simulink model "hydelcompleted_nosubsys"  (R2024b)
settings: Solver=VariableStepAuto  StartTime=0.0  StopTime=10.0  RelTol=1e-3
libraries: spsLoadFlowBusLib x3, spsThreePhaseParallelRLCLoadLib x2, spsThreePhaseVIMeasurementLib x2, spsDistributedParametersLineLib x1, spsExcitationSystemLib x1, spsHydraulicTurbineandGovernorLib x1, spsPower3phInstantaneousLib x1, spsSynchronousMachinepuStandardLib x1, spsThreePhaseTransformerTwoWindingsLib x1, sps_lib x1
settings Model: Creator=Ram  LastModifiedBy=Ram

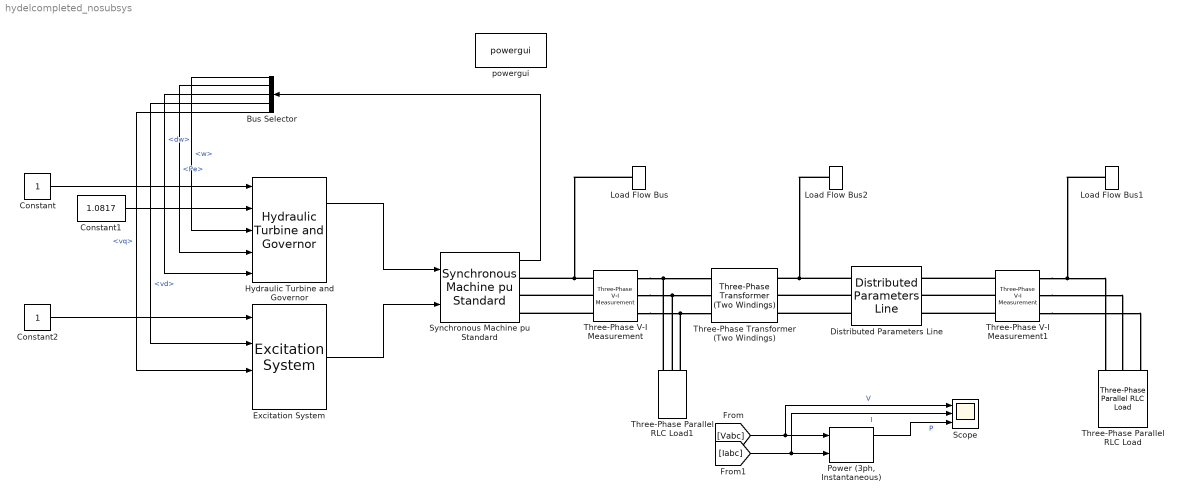
== system hydelcompleted_nosubsys ==
  Bus Selector : BusSelector  OutputSignals=w,Pe,dw,vd,vq
  Constant : Constant
  Constant1 : Constant  Value=1.0817
  Constant2 : Constant
  Distributed Parameters Line : spsDistributedParametersLineLib/Distributed Parameters Line  Phases=3  Length=100  Frequency=50  Resistance=[0.01273 0.3864]  Inductance="[0.9337e-3  4.1264e-3]"  Capacitance=[12.74e-9 7.751e-9]  x1=[-0.0006 -3.40260704829599e-09 112958.573096956 -396382.373244938;-0.00055 -3.37817671582999e-09 119170.741391489 -394559.196384513;-0.0005 -3.35291286880809e-09 125353.506088773 -392638.667946296;-0.00045 -3.32682174070653e-09 131505.341684135 -390621.261791942;-0.0004 -3.29990976912076e-09 137624.730304193 -388507.475686232;-0.00035 -3.27218359417706e-09 143710.162081371 -386297.831174258;-0.0003 -3.24365005689423e-09 149760.135526437 -383992.873452741;-0.00025 -3.21431619749565e-09 155773.157898971 -381593.171235508;-0.0002 -3.18418925367217e-09 161747.745575677 -379099.316613174;-0.00015 -3.1532766587964e-09 167682.424416446 -376511.92490705;-0.0001 -3.12158604008856e-09 173575.730128076 -373831.634517325;-5e-05 -3.08912521673463e-09 179426.208625566 -371059.106765545]  x2=[-0.0006 -3.5386891368581e-09 106068.858641917 -400380.951134164;-0.00055 -3.5176747746853e-09 112344.683835126 -398665.499910241;-0.0005 -3.49579247889795e-09 118592.789658648 -396851.683939575;-0.00045 -3.4730476486251e-09 124811.634485864 -394939.950754116;-0.0004 -3.44944589581327e-09 130999.683909868 -392930.772045422;-0.00035 -3.42499304384182e-09 137155.411122057 -390824.643548275;-0.0003 -3.39969512608608e-09 143277.297288852 -388622.084918367;-0.00025 -3.3735583844287e-09 149363.831926445 -386323.639604083;-0.0002 -3.3465892677196e-09 155413.513273489 -383929.874712411;-0.00015 -3.31879443018478e-09 161424.848661635 -381441.380869019;-0.0001 -3.2901807297845e-09 167396.354883826 -378858.772072529;-5e-05 -3.26075522652118e-09 173326.558560255 -376182.685543014]  x3=[-0.0006 -2.64139611004173e-12 190.415973613975 -1253.14025946932;-0.00055 -2.63703449038585e-12 210.07595415956 -1249.99473854659;-0.0005 -2.63202222192825e-12 229.684101606891 -1246.54080012619;-0.00045 -2.62636054137119e-12 249.235577938987 -1242.77929641575;-0.0004 -2.62005084564962e-12 268.725559121619 -1238.71115551002;-0.00035 -2.61309469158654e-12 288.149236293565 -1234.33738116191;-0.0003 -2.6054937955089e-12 307.501816953124 -1229.65905253478;-0.00025 -2.59725003282405e-12 326.778526140599 -1224.67732393622;-0.0002 -2.58836543755709e-12 345.974607616441 -1219.39342453322;-0.00015 -2.57884220184896e-12 365.085325034782 -1213.80865804889;-0.0001 -2.56868267541556e-12 384.10596311206 -1207.9244024408;-5e-05 -2.55788936496803e-12 403.031828790441 -1201.74210956096]  x4=[-0.0006 -7.19418612714017e-12 456.56208442296 -1723.39809180542;-0.00055 -7.1670537441911e-12 483.57572017421 -1716.01411492715;-0.0005 -7.13815299797357e-12 510.470040852406 -1708.20673724329;-0.00045 -7.10749101931428e-12 537.238410686349 -1699.97788510746;-0.0004 -7.07507537359763e-12 563.874224981325 -1691.32958886579;-0.00035 -7.04091405889918e-12 590.370911748719 -1682.26398235598;-0.0003 -7.00501550401215e-12 616.721933327548 -1672.78330238078;-0.00025 -6.96738856636781e-12 642.920787997537 -1662.88988815611;-0.0002 -6.92804252984998e-12 668.961011583318 -1652.58618073389;-0.00015 -6.88698710250445e-12 694.836179049369 -1641.87472239975;-0.0001 -6.84423241414356e-12 720.539906085297 -1630.75815604577;-5e-05 -6.79978901384694e-12 746.065850681068 -1619.23922451833]  x5=0.000565541566995743  V1=[2.409e-07 4.122e+05 4.122e+05;314.2 314.2 314.2;0.4186 0.3578 -1.213]  V2=[2.389e-07 4.142e+05 4.142e+05;314.2 314.2 314.2;0.3317 0.3391 -1.232]  I1=[1.745e-10 1268 1268;314.2 314.2 314.2;0.1145 0.2309 -1.34]  I2=[4.629e-10 1783 1783;314.2 314.2 314.2;0.3479 0.3391 -1.232]  nHarmo=1  Measurements=None  Decoupling=off  VsMag0=0  VrMag0=0  VsAngle0=0  VrAngle0=0  IsMag0=0  IrMag0=0  IsAngle0=0  IrAngle0=0
      settings: LibrarySourceBlock=sps_lib/Power Grid Elements/Distributed Parameters Line
  Excitation System : spsExcitationSystemLib/Excitation System  tr=20e-3  reg=[ 300, 0.001 ]  exc=[ 1, 0 ]  tgr=[ 0, 0 ]  damp=[ 0.001, 0.1 ]  sat=[ 0, 0 ]  lim=[ -11.5, 11.5, 0 ]  v0=[1 2.1744]
      settings: LibrarySourceBlock=sps_lib/Electrical Machines/Synchronous Machine Control/Excitation System
  Hydraulic Turbine and Governor : spsHydraulicTurbineandGovernorLib/Hydraulic Turbine and Governor  sm="[ 10/3  0.07 ]"  gate="[  0.01  0.97518  -0.1  0.1 ]"  reg="[  0.05  1.163  0.105  0  0.01  ]"  hyd="[  0  2.67  ]"  dref=0  po=1.0094
      settings: LibrarySourceBlock=|
      | sps_lib/Electrical Machines/Synchronous Machine Control/Hydraulic Turbine
      | and Governor
  Load Flow Bus : spsLoadFlowBusLib/Load Flow Bus  LConnTagsString=a  Phases=single  Connectors=on one side  ID=BUS_1  Vbase=13.8e3  Vref=1  Vangle=0  VLF=1  VLFb=1  VLFc=1  angleLF=0  angleLFb=0  angleLFc=0
  Load Flow Bus1 : spsLoadFlowBusLib/Load Flow Bus  LConnTagsString=a  Phases=single  Connectors=on one side  ID=BUS_3  Vbase=400e3  Vref=1  Vangle=0  VLF=1.036  VLFb=1  VLFc=1  angleLF=-4.321  angleLFb=0  angleLFc=0
  Load Flow Bus2 : spsLoadFlowBusLib/Load Flow Bus  LConnTagsString=a  Phases=single  Connectors=on one side  ID=BUS_2  Vbase=400e3  Vref=1  Vangle=0  VLF=1.031  VLFb=1  VLFc=1  angleLF=-3.252  angleLFb=0  angleLFc=0
  "Power (3ph, Instantaneous)" : spsPower3phInstantaneousLib/Power (3ph, Instantaneous)
  Scope : Scope  NumInputPorts=3
  Synchronous Machine pu Standard : spsSynchronousMachinepuStandardLib/Synchronous Machine pu Standard  PresetModel=No  MechanicalLoad=Mechanical power Pm  ShowDetailedParameters=on  RotorType=Salient-pole  Units=per unit standard parameters  MeasurementBus=on  NominalParameters=[100e6 13.8e3 50]  Reactances1=[ 1.81, 0.3, 0.23, 1.76, 0.65, 0.25, 0.15 ]  Reactances2=[2.24 0.17 0.12 1.02 0.13 0.08]  dAxisTimeConstants=Short-circuit  qAxisTimeConstants=Short-circuit  TimeConstants1="[ 4.4849  0.0681  0.1  ]"  TimeConstants2=[ 8.0, 0.03, 1.0, 0.07 ]  TimeConstants3="[  4.49  0.0681  0.0513  ]"  TimeConstants4=[ 8.0, 0.03, 0.3371, 0.0295 ]  TimeConstants5=[ 1.01, 0.053, 0.1 ]  TimeConstants6=[ 1.3201, 0.023, 1.0, 0.07 ]  TimeConstants7=[0.012 0.003 0.003]  TimeConstants8=[ 1.3201, 0.0231, 0.3371, 0.0295 ]  StatorResistance=0.037875  Mechanical=[0.1028 0.02056 12]  PolePairs=20  InitialConditions=[0 -21.9196 1.2258 1.2258 1.2258 28.0638 -91.9362 148.064 2.17443]  SetSaturation=on  Saturation=[0.6404,0.7127,0.8441,0.9214,0.9956,1.082,1.19,1.316,1.457;0.7,0.7698,0.8872,0.9466,0.9969,1.046,1.1,1.151,1.201]  LoadFlowParameters=[1,0,0,0,0]  TsPowergui=0  TsBlock=-1  IterativeModel=Trapezoidal non iterative  IterativeDiscreteModel=Trapezoidal non iterative  BusType=swing  Pref=0  Qref=0  Qmin=-Inf  Qmax=Inf  PLF=0  QLF=0
  Three-Phase Parallel RLC Load : spsThreePhaseParallelRLCLoadLib/Three-Phase Parallel RLC Load  LConnTagsString=A|B|C  Configuration=Y (grounded)  NominalVoltage=400e3  Vabc=[1e3 1e3 1e3]  Vabcp=[1e3 1e3 1e3]  NominalFrequency=50  UnbalancedPower=off  ActivePower=100000000  InductivePower=100  CapacitivePower=0  Pabc=[10e3 9e3 11e3]  QLabc=[100 90 110]  QCabc=[100 90 110]  Pabcp=[10e3 9e3 11e3]  QLabcp=[100 90 110]  QCabcp=[100 90 110]  Measurements=None  LoadType=constant Z
  Three-Phase Parallel RLC Load1 : spsThreePhaseParallelRLCLoadLib/Three-Phase Parallel RLC Load  LConnTagsString=A|B|C  Configuration=Y (grounded)  NominalVoltage=13.8e3  Vabc=[1e3 1e3 1e3]  Vabcp=[1e3 1e3 1e3]  NominalFrequency=50  UnbalancedPower=off  ActivePower=100  InductivePower=0  CapacitivePower=0  Pabc=[10e3 9e3 11e3]  QLabc=[100 90 110]  QCabc=[100 90 110]  Pabcp=[10e3 9e3 11e3]  QLabcp=[100 90 110]  QCabcp=[100 90 110]  Measurements=None  LoadType=constant Z
  Three-Phase Transformer (Two Windings) : spsThreePhaseTransformerTwoWindingsLib/Three-Phase Transformer (Two Windings)  Winding1Connection=Yg  Winding2Connection=Yg  CoreType=Three single-phase transformers  SetSaturation=off  Hysteresis=off  DataFile='hysteresis'  SetInitialFlux=off  Measurements=None  UNITS=pu  NominalPower=[ 250e6 , 50 ]  Winding1=[ 13.8e3 , 0.002 , 0.08 ]  Winding2=[ 400e3 , 0.002 , 0.08 ]  Rm=500  Lm=500  L0=0.5  Saturation=[ 0,0 ; 0.0024,1.2 ; 1.0,1.52 ]  InitialFluxes=[ 0.8 , -0.8 , 0.7 ]  BreakLoop=off  DiscreteSolver=Trapezoidal iterative  DataType=off  TransfoNumber=1
  Three-Phase V-I Measurement : spsThreePhaseVIMeasurementLib/Three-Phase V-I Measurement  VoltageMeasurement=phase-to-ground  SetLabelV=on  LabelV=Vabc  Vpu=off  VpuLL=off  CurrentMeasurement=yes  SetLabelI=on  LabelI=Iabc  Ipu=off  Pbase=100e6  Vbase=500e3  OutputType=Complex  PhasorSimulation=off  PSBequivalent=0
  Three-Phase V-I Measurement1 : spsThreePhaseVIMeasurementLib/Three-Phase V-I Measurement  VoltageMeasurement=phase-to-ground  SetLabelV=on  LabelV=Vabc1  Vpu=off  VpuLL=off  CurrentMeasurement=yes  SetLabelI=on  LabelI=Iabc1  Ipu=off  Pbase=100e6  Vbase=500e3  OutputType=Complex  PhasorSimulation=off  PSBequivalent=0
  powergui : sps_lib/powergui  Priority=1  SimulationMode=Discrete  SampleTime=50e-6  frequency=60  Iterations=50  frequencyindice=50  Pbase=100e6  ErrMax=1e-4  UnitsV=kV  UnitsW=MW  buscounter=0  FunctionMessages=off  echomessages=off  EnableUseOfTLC=off  CurrentSourceSwitches=off  DisableSnubberDevices=off  DisableRonSwitches=off  DisableVfSwitches=off  DisplayEquations=off  AutomaticDiscreteSolvers=off  SolverType=Tustin/Backward Euler (TBE)  Interpol=off  ExternalGateDelay=off  methode=off  Ts=100  x0status=blocks  SPID=on  SwTol=0  HookPort=off  NonlinearTolerance=1e-4  nMaxIteration=100  ContinueOnMaxIteration=off  RestoreLinks=warning  ResistiveCurrentMeasurement=off  Frange=[0:2:500]  Ylog=off  Xlog=on  ShowGrid=off  save=off  variable=ZData  structure=0  ZoomFFT=off  StartTime=0.0  cycles=1  DisplayStyle=1  fundamental=60  FreqAxis=off  MaxFrequency=1000  frequencyindicesteady=1  RmsSteady=1  display=off
  wires:
  [Vabc] -> Scope/1, "Power (3ph, Instantaneous)"/1  "V"
  [Iabc] -> Scope/2, "Power (3ph, Instantaneous)"/2  "I"
  Hydraulic Turbine and Governor/1 -> Synchronous Machine pu Standard/1
  Excitation System/1 -> Synchronous Machine pu Standard/2
  Synchronous Machine pu Standard/1 -> Bus Selector/1
  Bus Selector/1 -> Hydraulic Turbine and Governor/3  "<w>"
  Bus Selector/2 -> Hydraulic Turbine and Governor/4  "<Pe>"
  Bus Selector/3 -> Hydraulic Turbine and Governor/5  "<dw>"
  Bus Selector/4 -> Excitation System/2  "<vd>"
  Bus Selector/5 -> Excitation System/3  "<vq>"
  Constant/1 -> Hydraulic Turbine and Governor/1
  Constant1/1 -> Hydraulic Turbine and Governor/2
  Constant2/1 -> Excitation System/1
  "Power (3ph, Instantaneous)"/1 -> Scope/3  "P"
  connections:
  Three-Phase V-I Measurement/LConn3 -- Synchronous Machine pu Standard/RConn3
  Three-Phase V-I Measurement/LConn2 -- Synchronous Machine pu Standard/RConn2
  Three-Phase V-I Measurement/LConn1 -- Load Flow Bus/LConn1 -- Synchronous Machine pu Standard/RConn1
  Three-Phase V-I Measurement/RConn2 -- Three-Phase Parallel RLC Load1/LConn2 -- Three-Phase Transformer (Two Windings)/LConn2
  Three-Phase V-I Measurement/RConn1 -- Three-Phase Parallel RLC Load1/LConn1 -- Three-Phase Transformer (Two Windings)/LConn1
  Three-Phase V-I Measurement/RConn3 -- Three-Phase Parallel RLC Load1/LConn3 -- Three-Phase Transformer (Two Windings)/LConn3
  Distributed Parameters Line/LConn1 -- Load Flow Bus2/LConn1 -- Three-Phase Transformer (Two Windings)/RConn1
  Distributed Parameters Line/LConn2 -- Three-Phase Transformer (Two Windings)/RConn2
  Distributed Parameters Line/LConn3 -- Three-Phase Transformer (Two Windings)/RConn3
  Three-Phase V-I Measurement1/LConn3 -- Distributed Parameters Line/RConn3
  Three-Phase V-I Measurement1/LConn2 -- Distributed Parameters Line/RConn2
  Three-Phase V-I Measurement1/LConn1 -- Distributed Parameters Line/RConn1
  Three-Phase V-I Measurement1/RConn1 -- Load Flow Bus1/LConn1 -- Three-Phase Parallel RLC Load/LConn1
  Three-Phase V-I Measurement1/RConn2 -- Three-Phase Parallel RLC Load/LConn2
  Three-Phase V-I Measurement1/RConn3 -- Three-Phase Parallel RLC Load/LConn3
